simulink model "ZT_VehCtrl_18B_CAN"  (R2018b)
settings: Solver=FixedStepAuto  StartTime=0.0  StopTime=inf  FixedStep=0.005  RelTol=1e-3
InitFcn:
  | mbd_mpc_consistency_checks(bdroot(gcs));
values from neighbouring files (symbols this model uses):
  BatoverTempTh = single(80)    [VCU_INIT.m]
  BRS_PwrValid = single(5)    [VCU_INIT.m]
  BRSEnSpdTh1 = single(10)    [VCU_INIT.m]
  BRSEnSpdTh2 = single(20)    [VCU_INIT.m]
  MCUTempAlarmTh = single (60)    [VCU_INIT.m]
  mps2kmh = single(3.6)    [VCU_INIT.m]
  MtrPwrFac = single(1/9550)    [VCU_INIT.m]
  MtrTempAlarmTh = single (50)    [VCU_INIT.m]
  Padle1Signal1_Th = [PadleSignal1_min,PadleSignal1_max]    [VCU_INIT.m]
  Padle1Signal2_Th = [PadleSignal2_min,PadleSignal2_max]    [VCU_INIT.m]
  PadleSignal1_max = 3.84    [VCU_INIT.m]
  PadleSignal1_min = 0.75    [VCU_INIT.m]
  PadleSignal2_max = 1.92    [VCU_INIT.m]
  PadleSignal2_min = 0.375    [VCU_INIT.m]
  PadleValid = 0.05    [VCU_INIT.m]
  PwrLimFactor = single(0.5)    [VCU_INIT.m]
  Ratio = single(1)    [VCU_INIT.m]
  rpm2mps = single(2*pi/60 * WhlRadius/Ratio)    [VCU_INIT.m]
  SOCLowTh = single(20)    [VCU_INIT.m]
  VehPwrBackwardMax = VehPwrMax * single(0.3)    [VCU_INIT.m]
  VehPwrMax = single(MtrPwrMax * 4)    [VCU_INIT.m]
  VehTrqBackwardMax = VehTrqMax * single(0.3)    [VCU_INIT.m]
  VehTrqMax = single(MtrTrqMax * Ratio *4)    [VCU_INIT.m]
  WhlRadius = single(1)    [VCU_INIT.m]
undefined symbols (not defined in the file or in its folder): Delay_Charge, Delay_Discharge, fifo_0_vect, fifo_1_vect, LQFP, pts1_fifo_0_vect, pts1_fifo_1_vect, pts2_fifo_0_vect, pts2_fifo_1_vect, pts3_fifo_0_vect, pts3_fifo_1_vect, pts4_fifo_0_vect, pts4_fifo_1_vect
libraries: mbd_mpc574x_ec_toolbox x157, canmsglib x74, simulink x38
(part 5 of 12)

== system ZT_VehCtrl_18B_CAN/VehCtrl/EnergyManage ==
  BMS : Inport
  OBC : Inport  Port=2
  HVC : Inport  Port=3
  PDU : Inport  Port=4
  DCDC : Inport  Port=5
  BRS : Inport  Port=6
  DAQ : Inport  Port=7
  Fault : Inport  Port=8
  DrvMtrPwrFb : Inport  Port=9
  VehSpdFb : Inport  Port=10
  Bus Creator : BusCreator  Inputs=2
  Bus Creator1 : BusCreator  Inputs=2
  Bus Creator{4..5,7..10} (6 alike) : BusCreator  Inputs=1
  Bus Creator2 : BusCreator  Inputs=3
  Bus Creator3 : BusCreator  Inputs=3
  Bus Creator6 : BusCreator  Inputs=2
  Bus Selector1 : BusSelector  OutputSignals=BMS_Information2.BMS_ReadySt,BMS_Information2.BMS_PrechargeStatus,BMS Power Infor.BMS_BatteryPower
  Bus Selector2 : BusSelector  OutputSignals=OBC_Charger Status.OBC_StartSt
  Bus Selector4 : BusSelector  OutputSignals=ShutDown,NonBRS,NonOBC
  Bus Selector5 : BusSelector  OutputSignals=ChargeEnSw,AccPadle
  Chart : Stateflow chart  TreatAsAtomicUnit=on
  Data Store Write : DataStoreWrite  DataStoreName=EnergyFlag
  "BMS_OUT " : Outport
  "DCDC_OUT " : Outport  Port=2
  BRS_OUT : Outport  Port=3
  HVC_OUT : Outport  Port=4
  MCU1_OUT : Outport  Port=5
  MCU2_OUT : Outport  Port=6
  ACU_OUT : Outport  Port=7
  PDU_OUT : Outport  Port=8
  TM_OUT : Outport  Port=9
  ISG_OUT : Outport  Port=10
  Ready : Outport  Port=11
  wires:
  BMS/1 -> Bus Selector1/1
  Bus Selector1/1 -> Chart/1(BMS_ReadySt)  "<BMS_ReadySt>"
  OBC/1 -> Bus Selector2/1
  Bus Selector2/1 -> Chart/4(OBC_Start)  "<OBC_StartSt>"
  Bus Selector1/2 -> Chart/2(BMS_PrechargeStatus)  "<BMS_PrechargeStatus>"
  Bus Creator/1 -> "BMS_OUT "/1
  Bus Selector1/3 -> Chart/3(BMS_BatteryPower)  "<BMS_BatteryPower>"
  Chart/1(VCU_PowerOnReq) -> Bus Creator/1  "VCU_PowerOnReq"
  Chart/2(VCU_UrgencyCutOffPowerReq) -> Bus Creator/2  "VCU_UrgencyCutOffPowerReq"
  Chart/11(DcdcCmd) -> Bus Creator1/1  "DcdcCmd"
  Chart/12(DcacEpsCmd) -> Bus Creator1/2  "DcacEpsCmd"
  Bus Creator1/1 -> ACU_OUT/1
  Chart/4(MaxChargePowerLimit) -> Bus Creator2/1  "MaxChargePowerLimit"
  Chart/5(BRS_PowerReq) -> Bus Creator2/2  "BRS_PowerReq"
  Chart/6(OnOffCmd) -> Bus Creator2/3  "OnOffCmd"
  Bus Creator2/1 -> BRS_OUT/1
  Chart/15(VCU_DCCpstRlyCtl) -> Bus Creator3/3  "VCU_DCCpstRlyCtl"
  Chart/14(VCU_HghVtgCtl) -> Bus Creator3/2  "VCU_HghVtgCtl"
  Chart/13(VCU_ShrRlyCtl) -> Bus Creator3/1  "VCU_ShrRlyCtl"
  Chart/9(VCU2OilMotor_ActiveDisCharge) -> Bus Creator5/1  "VCU2OilMotor_ActiveDisCharge"
  Chart/10(VCU2DrvMotor_ActiveDisCharge) -> Bus Creator10/1  "VCU2DrvMotor_ActiveDisCharge"
  Chart/18(TM_Discharge) -> Bus Creator8/1  "TM_Discharge"
  Chart/19(ISG_Discharge) -> Bus Creator9/1  "ISG_Discharge"
  Bus Creator3/1 -> PDU_OUT/1
  Bus Creator6/1 -> HVC_OUT/1
  Chart/7(EDrv1_PowOnCmd) -> Bus Creator6/1  "EDrv1_PowOnCmd"
  Chart/8(EDrv2_PowOnCmd) -> Bus Creator6/2  "EDrv2_PowOnCmd"
  Fault/1 -> Bus Selector4/1
  Bus Selector4/1 -> Chart/8(ShutDown)  "<ShutDown>"
  Bus Selector4/2 -> Chart/9(NonBRS)  "<NonBRS>"
  Bus Selector4/3 -> Chart/10(NonOBC)  "<NonOBC>"
  Chart/16(Ready) -> Bus Creator7/1  "Ready"
  Chart/17(Flag) -> Data Store Write/1  "Flag"
  DAQ/1 -> Bus Selector5/1
  Bus Selector5/1 -> Chart/11(ChargeSig)  "<ChargeEnSw>"
  DrvMtrPwrFb/1 -> Chart/6(PwrCupReq)
  Bus Selector5/2 -> Chart/12(AccPadle)  "<AccPadle>"
  VehSpdFb/1 -> Chart/13(VehSpdFb)
  Chart/3(VCU_DCDC1_En) -> Bus Creator4/1  "VCU_DCDC1_En"
  Bus Creator4/1 -> "DCDC_OUT "/1
  Bus Creator5/1 -> MCU1_OUT/1
  Bus Creator7/1 -> Ready/1
  Bus Creator8/1 -> TM_OUT/1
  Bus Creator9/1 -> ISG_OUT/1
  Bus Creator10/1 -> MCU2_OUT/1

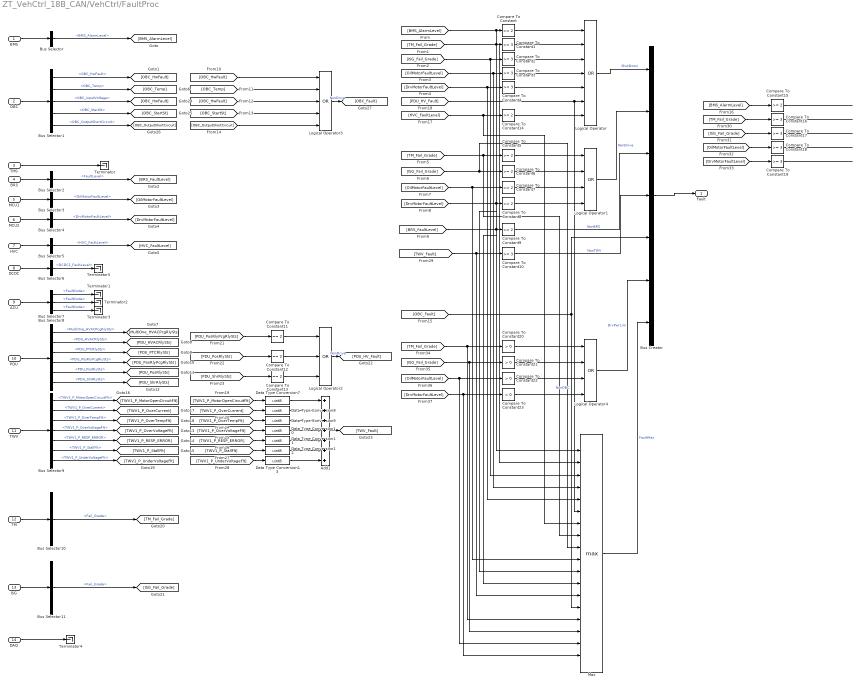
== system ZT_VehCtrl_18B_CAN/VehCtrl/FaultProc ==
  "BMS " : Inport
  "OBC " : Inport  Port=2
  "TMS " : Inport  Port=3
  "BRS " : Inport  Port=4
  "MCU1 " : Inport  Port=5
  MCU2 : Inport  Port=6
  HVC : Inport  Port=7
  DCDC : Inport  Port=8
  ACU : Inport  Port=9
  PDU : Inport  Port=10
  TWV : Inport  Port=11
  TM : Inport  Port=12
  ISG : Inport  Port=13
  DAQ : Inport  Port=14
  Add1 : Sum  Inputs=+++++++
  Bus Creator : BusCreator  Inputs=7
  Bus Selector : BusSelector  OutputSignals=BMS_Information2.BMS_AlarmLevel
  Bus Selector1 : BusSelector  OutputSignals=OBC_Charger Status.OBC_HwFault,OBC_Charger Status.OBC_Temp,OBC_Charger Status.OBC_InputVoltage,OBC_Charger Status.OBC_StartSt,OBC_Charger Status.OBC_OutputShortCircuit
  Bus Selector10 : BusSelector  OutputSignals=TM_MCU_STATUS_2.Fail_Grade
  Bus Selector11 : BusSelector  OutputSignals=ISG_MCU_STATUS_2.Fail_Grade
  Bus Selector2 : BusSelector  OutputSignals=BRS2VCU1.FaultLevel
  Bus Selector3 : BusSelector  OutputSignals=MCU1Msg2.OilMotorFaultLevel
  Bus Selector4 : BusSelector  OutputSignals=MCU2Msg2.DrvMotorFaultLevel
  Bus Selector5 : BusSelector  OutputSignals=HVC4_RlySt.HVC_FaultLevel
  Bus Selector6 : BusSelector  OutputSignals=DCDC1_2.DCDC1_FaultLevel
  Bus Selector7 : BusSelector  OutputSignals=ACU1.FaultCode,ACU2.FaultCode,ACU3.FaultCode
  Bus Selector8 : BusSelector  OutputSignals=PDU_RelaySts.MultiOne_HVACPcgRlySts,PDU_RelaySts.PDU_HVACRlySts,PDU_RelaySts.PDU_PTCRlySts,PDU_RelaySts.PDU_PosRlyPcgRlySts,PDU_RelaySts.PDU_PosRlySts,PDU_RelaySts.PDU_ShrRlySts
  Bus Selector9 : BusSelector  OutputSignals=TWV.TWV1_P_MotorOpenCircuitFlt,TWV.TWV1_P_OverCurrent,TWV.TWV1_P_OverTempFlt,TWV.TWV1_P_OverVoltageFlt,TWV.TWV1_P_RESP_ERROR,TWV.TWV1_P_StallFlt,TWV.TWV1_P_UnderVoltageFlt
  Compare To Constant{,5..9,14..15} (8 alike) : simulink/Logic and Bit Operations/Compare To Constant  relop=>=  const=2  OutDataTypeStr=boolean
  Compare To Constant{1..4,10,16..19} (9 alike) : simulink/Logic and Bit Operations/Compare To Constant  relop=>=  const=3  OutDataTypeStr=boolean
  Compare To Constant11 : simulink/Logic and Bit Operations/Compare To Constant  relop===  const=2  OutDataTypeStr=boolean
  Compare To Constant12 : simulink/Logic and Bit Operations/Compare To Constant  relop===  const=2  OutDataTypeStr=boolean
  Compare To Constant13 : simulink/Logic and Bit Operations/Compare To Constant  relop===  const=2  OutDataTypeStr=boolean
  Compare To Constant{20..23} (4 alike) : simulink/Logic and Bit Operations/Compare To Constant  relop=>  const=0  OutDataTypeStr=boolean
  Data Type Conversion{7..13} (7 alike) : DataTypeConversion  OutDataTypeStr=uint8
  Logical Operator : Logic  Operator=OR  Inputs=7  AllPortsSameDT=off  OutDataTypeStr=boolean
  Logical Operator1 : Logic  Operator=OR  Inputs=4  AllPortsSameDT=off  OutDataTypeStr=boolean
  Logical Operator2 : Logic  Operator=OR  Inputs=3  AllPortsSameDT=off  OutDataTypeStr=boolean
  Logical Operator3 : Logic  Operator=OR  Inputs=5  AllPortsSameDT=off  OutDataTypeStr=boolean
  Logical Operator4 : Logic  Operator=OR  Inputs=4  AllPortsSameDT=off  OutDataTypeStr=boolean
  Max : MinMax  Function=max  Inputs=18
  Terminator{,1..5} (6 alike) : Terminator
  "Fault " : Outport
  wires:
  "BMS "/1 -> Bus Selector/1
  Bus Selector/1 -> [BMS_AlarmLevel]  "<BMS_AlarmLevel>"
  "OBC "/1 -> Bus Selector1/1
  Bus Selector1/1 -> [OBC_HwFault]  "<OBC_HwFault>"
  "TMS "/1 -> Terminator/1
  "BRS "/1 -> Bus Selector2/1
  "MCU1 "/1 -> Bus Selector3/1
  Bus Selector3/1 -> [OilMotorFaultLevel]  "<OilMotorFaultLevel>"
  Bus Selector2/1 -> [BRS_FaultLevel]  "<FaultLevel>"
  MCU2/1 -> Bus Selector4/1
  Bus Selector4/1 -> [DrvMotorFaultLevel]  "<DrvMotorFaultLevel>"
  HVC/1 -> Bus Selector5/1
  Bus Selector5/1 -> [HVC_FaultLevel]  "<HVC_FaultLevel>"
  DCDC/1 -> Bus Selector6/1
  Bus Selector6/1 -> Terminator5/1  "<DCDC1_FaultLevel>"
  ACU/1 -> Bus Selector7/1
  Bus Selector7/1 -> Terminator1/1  "<FaultCode>"
  Bus Selector7/2 -> Terminator2/1  "<FaultCode>"
  Bus Selector7/3 -> Terminator3/1  "<FaultCode>"
  PDU/1 -> Bus Selector8/1
  TWV/1 -> Bus Selector9/1
  TM/1 -> Bus Selector10/1
  ISG/1 -> Bus Selector11/1
  DAQ/1 -> Terminator4/1
  Bus Selector8/1 -> [MultiOne_HVACPcgRlySts]  "<MultiOne_HVACPcgRlySts>"
  Bus Selector8/2 -> [PDU_HVACRlySts]  "<PDU_HVACRlySts>"
  Bus Selector8/3 -> [PDU_PTCRlySts]  "<PDU_PTCRlySts>"
  Bus Selector8/4 -> [PDU_PosRlyPcgRlySts]  "<PDU_PosRlyPcgRlySts>"
  Bus Selector8/5 -> [PDU_PosRlySts]  "<PDU_PosRlySts>"
  Bus Selector8/6 -> [PDU_ShrRlySts]  "<PDU_ShrRlySts>"
  Bus Selector9/1 -> [TWV1_P_MotorOpenCircuitFlt]  "<TWV1_P_MotorOpenCircuitFlt>"
  Bus Selector9/2 -> [TWV1_P_OverCurrent]  "<TWV1_P_OverCurrent>"
  Bus Selector9/3 -> [TWV1_P_OverTempFlt]  "<TWV1_P_OverTempFlt>"
  Bus Selector9/4 -> [TWV1_P_OverVoltageFlt]  "<TWV1_P_OverVoltageFlt>"
  Bus Selector9/5 -> [TWV1_P_RESP_ERROR]  "<TWV1_P_RESP_ERROR>"
  Bus Selector9/6 -> [TWV1_P_StallFlt]  "<TWV1_P_StallFlt>"
  Bus Selector9/7 -> [TWV1_P_UnderVoltageFlt]  "<TWV1_P_UnderVoltageFlt>"
  Bus Selector10/1 -> [TM_Fail_Grade]  "<Fail_Grade>"
  Bus Selector11/1 -> [ISG_Fail_Grade]  "<Fail_Grade>"
  [BMS_AlarmLevel] -> Max/1, Compare To Constant/1
  [TM_Fail_Grade] -> Max/2, Compare To Constant1/1
  [ISG_Fail_Grade] -> Compare To Constant2/1, Max/3
  [DrvMotorFaultLevel] -> Compare To Constant4/1, Max/5
  [OilMotorFaultLevel] -> Compare To Constant3/1, Max/4
  Compare To Constant/1 -> Logical Operator/1
  Compare To Constant1/1 -> Logical Operator/2
  Compare To Constant2/1 -> Logical Operator/3
  Compare To Constant3/1 -> Logical Operator/4
  Compare To Constant4/1 -> Logical Operator/5
  Logical Operator/1 -> Bus Creator/1  "ShutDown"
  Bus Creator/1 -> "Fault "/1
  Compare To Constant8/1 -> Logical Operator1/4
  Compare To Constant7/1 -> Logical Operator1/3
  Compare To Constant6/1 -> Logical Operator1/2
  [OilMotorFaultLevel] -> Max/10, Compare To Constant7/1
  [DrvMotorFaultLevel] -> Max/11, Compare To Constant8/1
  [ISG_Fail_Grade] -> Max/9, Compare To Constant6/1
  [TM_Fail_Grade] -> Compare To Constant5/1, Max/8
  Compare To Constant5/1 -> Logical Operator1/1
  Logical Operator1/1 -> Bus Creator/2  "NonDrive"
  [BRS_FaultLevel] -> Max/12, Compare To Constant9/1
  Compare To Constant9/1 -> Bus Creator/3  "NonBRS"
  Compare To Constant10/1 -> Bus Creator/4  "NonTWV"
  [PDU_PosRlyPcgRlySts] -> Compare To Constant11/1
  [PDU_PosRlySts] -> Compare To Constant12/1
  [PDU_ShrRlySts] -> Compare To Constant13/1
  Compare To Constant11/1 -> Logical Operator2/1
  Compare To Constant12/1 -> Logical Operator2/2
  Compare To Constant13/1 -> Logical Operator2/3
  Logical Operator2/1 -> [PDU_HV_Fault]  "NonDrive"
  [PDU_HV_Fault] -> Max/6, Logical Operator/6
  [HVC_FaultLevel] -> Compare To Constant14/1, Max/7
  Compare To Constant14/1 -> Logical Operator/7
  Data Type Conversion13/1 -> Add1/7
  Data Type Conversion12/1 -> Add1/6
  Data Type Conversion11/1 -> Add1/5
  Data Type Conversion10/1 -> Add1/4
  Data Type Conversion9/1 -> Add1/3
  Data Type Conversion8/1 -> Add1/2
  Data Type Conversion7/1 -> Add1/1
  [TWV1_P_OverCurrent] -> Data Type Conversion8/1
  [TWV1_P_OverTempFlt] -> Data Type Conversion9/1
  [TWV1_P_OverVoltageFlt] -> Data Type Conversion10/1
  [TWV1_P_RESP_ERROR] -> Data Type Conversion11/1
  [TWV1_P_StallFlt] -> Data Type Conversion12/1
  [TWV1_P_UnderVoltageFlt] -> Data Type Conversion13/1
  [TWV1_P_MotorOpenCircuitFlt] -> Data Type Conversion7/1
  Add1/1 -> [TWV_Fault]
  [TWV_Fault] -> Compare To Constant10/1, Max/13
  Bus Selector1/2 -> [OBC_Temp]  "<OBC_Temp>"
  Bus Selector1/3 -> [OBC_HwFault]  "<OBC_InputVoltage>"
  Bus Selector1/4 -> [OBC_StartSt]  "<OBC_StartSt>"
  Bus Selector1/5 -> [OBC_OutputShortCircuit]  "<OBC_OutputShortCircuit>"
  [OBC_HwFault] -> Logical Operator3/1
  [OBC_Temp] -> Logical Operator3/2
  [OBC_HwFault] -> Logical Operator3/3
  [OBC_StartSt] -> Logical Operator3/4
  [OBC_OutputShortCircuit] -> Logical Operator3/5
  Logical Operator3/1 -> [OBC_Fault]  "NonDrive"
  [OBC_Fault] -> Bus Creator/5, Max/14  "NonOBC"
  Compare To Constant19/1 -> ?
  Compare To Constant18/1 -> ?
  Compare To Constant17/1 -> ?
  Compare To Constant16/1 -> ?
  Compare To Constant15/1 -> ?
  [OilMotorFaultLevel] -> Compare To Constant18/1
  [DrvMotorFaultLevel] -> Compare To Constant19/1
  [ISG_Fail_Grade] -> Compare To Constant17/1
  [TM_Fail_Grade] -> Compare To Constant16/1
  [BMS_AlarmLevel] -> Compare To Constant15/1
  Compare To Constant20/1 -> Logical Operator4/1
  [TM_Fail_Grade] -> Compare To Constant20/1, Max/15
  [ISG_Fail_Grade] -> Compare To Constant21/1, Max/16
  [DrvMotorFaultLevel] -> Compare To Constant23/1, Max/18
  [OilMotorFaultLevel] -> Max/17, Compare To Constant22/1
  Compare To Constant21/1 -> Logical Operator4/2
  Compare To Constant22/1 -> Logical Operator4/3
  Compare To Constant23/1 -> Logical Operator4/4
  Logical Operator4/1 -> Bus Creator/6  "DrvPwrLim"
  Max/1 -> Bus Creator/7  "FaultMax"

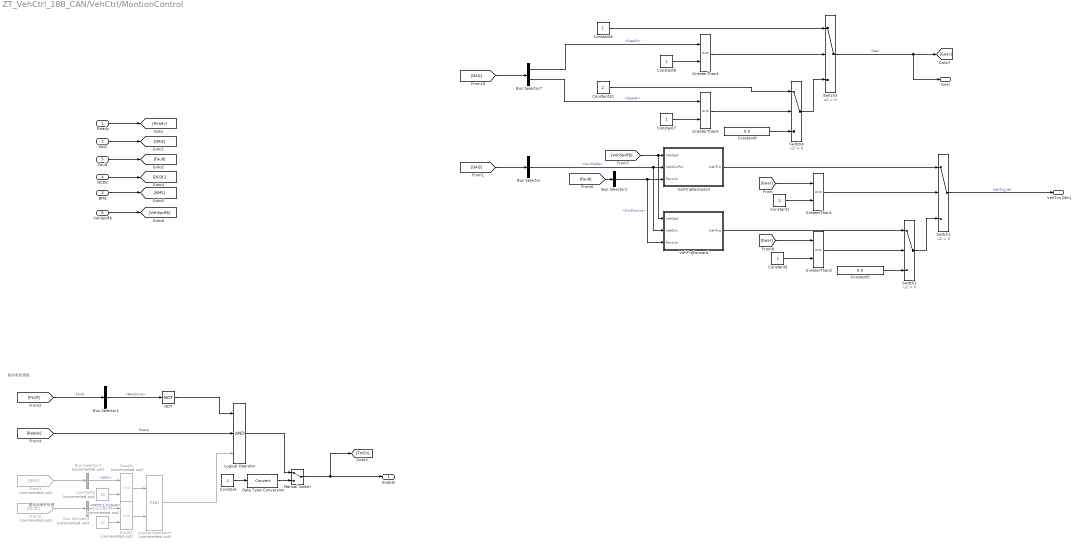
== system ZT_VehCtrl_18B_CAN/VehCtrl/MontionControl ==
  note: 驱动电机使能
  note: 蓄电池保护处理
  Ready : Inport
  DAQ : Inport  Port=2
  BMS : Inport  Port=3
  DCDC : Inport  Port=4
  Fault : Inport  Port=5
  VehSpdFb : Inport  Port=6
  Bus Selector : BusSelector  OutputSignals=AccPadle
  Bus Selector1 : BusSelector  OutputSignals=NonDrive
  Bus Selector2 : BusSelector  OutputSignals=DrvPwrLim
  Bus Selector3 : BusSelector  Commented=on  OutputSignals=BMS_Information1.SOC
  Bus Selector4 : BusSelector  Commented=on  OutputSignals=DCDC1_1.DCDC1_OutVolt
  Bus Selector7 : BusSelector  OutputSignals=GearD,GearR
  Constant : Constant
  Constant1 : Constant  Value=2  OutDataTypeStr=single
  Constant10 : Constant  Value=2  OutDataTypeStr=single
  Constant2 : Constant  Commented=on  Value=30  OutDataTypeStr=boolean
  Constant3 : Constant  OutDataTypeStr=single
  Constant4 : Constant  Commented=on  Value=22  OutDataTypeStr=boolean
  Constant5 : Constant  Value=0.0  OutDataTypeStr=single
  Constant6 : Constant  OutDataTypeStr=boolean
  Constant7 : Constant  OutDataTypeStr=boolean
  Constant8 : Constant  Value=0.0  OutDataTypeStr=single
  Constant9 : Constant  OutDataTypeStr=int8
  Data Type Conversion : DataTypeConversion
  Equal1 : RelationalOperator  Commented=on  OutDataTypeStr=boolean  RndMeth=Simplest
  Equal2 : RelationalOperator  Commented=on  OutDataTypeStr=boolean  RndMeth=Simplest
  From3 : From  Commented=on  GotoTag=BMS
  From5 : From  Commented=on  GotoTag=DCDC
  GreaterThan{1..2,4..5} (4 alike) : RelationalOperator  Operator===  OutDataTypeStr=boolean  RndMeth=Simplest
  Logical Operator : Logic  Inputs=3  AllPortsSameDT=off  OutDataTypeStr=boolean
  Logical Operator1 : Logic  Commented=on  AllPortsSameDT=off  OutDataTypeStr=boolean
  Manual Switch : ManualSwitch
  NOT : Logic  Operator=NOT  IconShape=distinctive  AllPortsSameDT=off  OutDataTypeStr=boolean
  Switch{1..4} (4 alike) : Switch  Criteria=u2 > Threshold
  VehTrqBackward : Subsystem
  VehTrqForward : Subsystem
  Enable : Outport
  VehTrq [Nm] : Outport  Port=2
  Gear : Outport  Port=3
  wires:
  Ready/1 -> [Ready]
  DAQ/1 -> [DAQ]
  [DAQ] -> Bus Selector/1
  Fault/1 -> [Fault]
  Bus Selector/1 -> VehTrqForward/2(VehDrv), VehTrqBackward/2(VehDrvPct)  "<AccPadle>"
  [Fault] -> Bus Selector1/1  "Fault"
  [Ready] -> Logical Operator/2  "Ready"
  Bus Selector4/1 -> Equal2/1  "<DCDC1_OutVolt>"
  Logical Operator/1 -> Manual Switch/1
  Equal2/1 -> Logical Operator1/2
  Data Type Conversion/1 -> Manual Switch/2
  Constant4/1 -> Equal2/2
  From5/1 -> Bus Selector4/1
  From3/1 -> Bus Selector3/1
  Bus Selector3/1 -> Equal1/1  "<SOC>"
  Logical Operator1/1 -> Logical Operator/3
  Manual Switch/1 -> [TmEn], Enable/1
  Equal1/1 -> Logical Operator1/1
  NOT/1 -> Logical Operator/1
  Constant/1 -> Data Type Conversion/1
  Bus Selector1/1 -> NOT/1  "<NonDrive>"
  Constant2/1 -> Equal1/2
  BMS/1 -> [BMS]
  DCDC/1 -> [DCDC]
  VehTrqForward/1(VehTrq) -> Switch2/1
  GreaterThan1/1 -> Switch1/2
  VehTrqBackward/1(VehTrq) -> Switch1/1
  Constant5/1 -> Switch2/3
  GreaterThan2/1 -> Switch2/2
  Constant1/1 -> GreaterThan1/2
  Switch2/1 -> Switch1/3
  Constant3/1 -> GreaterThan2/2
  Switch1/1 -> VehTrq [Nm]/1  "VehTrq_ter"
  [Fault] -> Bus Selector2/1
  Bus Selector2/1 -> VehTrqForward/3(PwrLim), VehTrqBackward/3(PwrLim)  "<DrvPwrLim>"
  VehSpdFb/1 -> [VehSpdFb]
  [VehSpdFb] -> VehTrqForward/1(VehSpd), VehTrqBackward/1(VehSpd)
  [DAQ] -> Bus Selector7/1
  Switch3/1 -> Gear/1, [Gear]  "Gear"
  Constant7/1 -> GreaterThan5/2
  Switch4/1 -> Switch3/3
  Constant6/1 -> GreaterThan4/2
  GreaterThan5/1 -> Switch4/2
  Constant8/1 -> Switch4/3
  Constant9/1 -> Switch3/1
  GreaterThan4/1 -> Switch3/2
  Constant10/1 -> Switch4/1
  Bus Selector7/1 -> GreaterThan4/1  "<GearD>"
  Bus Selector7/2 -> GreaterThan5/1  "<GearR>"
  [Gear] -> GreaterThan1/1
  [Gear] -> GreaterThan2/1

== system ZT_VehCtrl_18B_CAN/VehCtrl/SpdCalc ==
  MCU2 : Inport
  TM : Inport  Port=2
  MCU1 : Inport  Port=3
  ISG : Inport  Port=4
  Abs{1..4} (4 alike) : Abs
  Add{,1..3} (4 alike) : Sum
  Bus Selector : BusSelector  OutputSignals=MCU2Msg1.DrvMotorSpd,MCU2Msg1.DrvMotorTrq
  Bus Selector1 : BusSelector  OutputSignals=TM_MCU_STATUS_1.Motor_Speed,TM_MCU_STATUS_1.Motor_Torque
  Bus Selector2 : BusSelector  OutputSignals=MCU1Msg1.OilMotorSpd,MCU1Msg1.OilMotorTrq
  Bus Selector3 : BusSelector  OutputSignals=ISG_MCU_STATUS_1.Motor_Speed,ISG_MCU_STATUS_1.Motor_Torque
  Constant : Constant  Value=rpm2mps
  Gain : Gain  Gain=0.5
  Gain1 : Gain  Gain=MtrPwrFac
  Gain2 : Gain  Gain=MtrPwrFac
  Gain3 : Gain  Gain=Ratio
  Product{,1..4} (5 alike) : Product
  VehSpdFb : Outport
  "VehTrqFb " : Outport  Port=2
  "DrvMtrPwrFb " : Outport  Port=3
  "OilMtrPwrFb " : Outport  Port=4
  wires:
  MCU2/1 -> Bus Selector/1
  TM/1 -> Bus Selector1/1
  MCU1/1 -> Bus Selector2/1
  ISG/1 -> Bus Selector3/1
  Bus Selector1/1 -> Abs1/1  "<Motor_Speed>"
  Bus Selector3/1 -> Abs3/1  "<Motor_Speed>"
  Bus Selector/2 -> Add2/1, Product1/2  "<DrvMotorTrq>"
  Abs1/1 -> Product2/2, Add/2
  Add/1 -> Gain/1
  Product/1 -> VehSpdFb/1
  Gain/1 -> Product/1
  Constant/1 -> Product/2
  Abs2/1 -> Product1/1, Add/1
  Product1/1 -> Add1/1
  Product2/1 -> Add1/2
  Bus Selector1/2 -> Add2/2, Product2/1  "<Motor_Torque>"
  Add1/1 -> Gain1/1
  Gain1/1 -> "DrvMtrPwrFb "/1
  Add2/1 -> Gain3/1
  Bus Selector/1 -> Abs2/1  "<DrvMotorSpd>"
  Bus Selector2/1 -> Abs4/1  "<OilMotorSpd>"
  Bus Selector2/2 -> Product3/2  "<OilMotorTrq>"
  Bus Selector3/2 -> Product4/2  "<Motor_Torque>"
  Add3/1 -> Gain2/1
  Abs3/1 -> Product4/1
  Product3/1 -> Add3/1
  Gain2/1 -> "OilMtrPwrFb "/1
  Product4/1 -> Add3/2
  Abs4/1 -> Product3/1
  Gain3/1 -> "VehTrqFb "/1

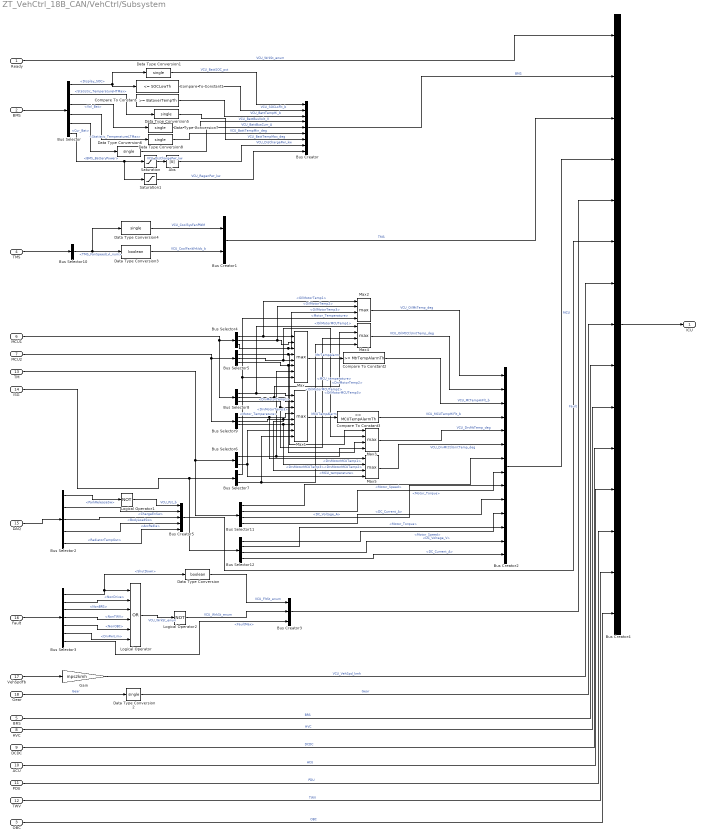
== system ZT_VehCtrl_18B_CAN/VehCtrl/Subsystem ==
  Ready : Inport
  BMS : Inport  Port=2
  OBC : Inport  Port=3
  TMS : Inport  Port=4
  BRS : Inport  Port=5
  MCU1 : Inport  Port=6
  MCU2 : Inport  Port=7
  HVC : Inport  Port=8
  DCDC : Inport  Port=9
  ACU : Inport  Port=10
  PDU : Inport  Port=11
  TWV : Inport  Port=12
  TM : Inport  Port=13
  ISG : Inport  Port=14
  DAQ : Inport  Port=15
  Fault : Inport  Port=16
  VehSpdFb : Inport  Port=17
  Gear : Inport  Port=18
  Abs : Abs
  Bus Creator : BusCreator  Inputs=9
  Bus Creator1 : BusCreator  Inputs=2
  Bus Creator2 : BusCreator  Inputs=14
  Bus Creator3 : BusCreator  Inputs=3
  Bus Creator4 : BusCreator  Inputs=15
  Bus Creator5 : BusCreator  Inputs=5
  Bus Selector : BusSelector  OutputSignals=BMS_Information1.Display_SOC,BMS Statistic_Temperature of Battery.Statistic_TemperatureHTMax,BMS_Information1.Vol_Bat,BMS Statistic_Temperature of Battery.Statistic_TemperatureLTMax,BMS_Information1.Cur_Bat,BMS Power Infor.BMS_BatteryPower
  Bus Selector10 : BusSelector  OutputSignals=TMS2VCU.TMS_FanSpeedLvl_num
  Bus Selector11 : BusSelector  OutputSignals=TM_MCU_STATUS_1.Motor_Speed,TM_MCU_STATUS_1.Motor_Torque,TM_MCU_STATUS_3.DC_Voltage_A,TM_MCU_STATUS_3.DC_Current_A
  Bus Selector12 : BusSelector  OutputSignals=ISG_MCU_STATUS_1.Motor_Speed,ISG_MCU_STATUS_1.Motor_Torque,ISG_MCU_STATUS_3.DC_Voltage_V,ISG_MCU_STATUS_3.DC_Current_A
  Bus Selector2 : BusSelector  OutputSignals=ParkReleaseSw,ChargeEnSw,BodyLoadSw,AccPadle,RadiatorTempOut
  Bus Selector3 : BusSelector  OutputSignals=ShutDown,NonDrive,NonBRS,NonTWV,NonOBC,DrvPwrLim,FaultMax
  Bus Selector4 : BusSelector  OutputSignals=MCU1Msg3.OilMotorTemp1,MCU1Msg3.OilMotorTemp2,MCU1Msg3.OilMotorTemp3
  Bus Selector5 : BusSelector  OutputSignals=MCU2Msg3.DrvMotorTemp1,MCU2Msg3.DrvMotorTemp2,MCU2Msg3.DrvMotorTemp3
  Bus Selector6 : BusSelector  OutputSignals=TM_MCU_STATUS_2.Motor_Temperature,TM_MCU_STATUS_2.MCU_temperature
  Bus Selector7 : BusSelector  OutputSignals=ISG_MCU_STATUS_2.Motor_Temperature,ISG_MCU_STATUS_2.MCU_temperature
  Bus Selector8 : BusSelector  OutputSignals=MCU1Msg3.OilMotorMCUTemp1,MCU1Msg3.OilMotorMCUTemp2,MCU1Msg3.OilMotorMCUTemp3
  Bus Selector9 : BusSelector  OutputSignals=MCU2Msg3.DrvMotorMCUTemp1,MCU2Msg3.DrvMotorMCUTemp2,MCU2Msg3.DrvMotorMCUTemp3
  Compare To Constant : simulink/Logic and Bit Operations/Compare To Constant  relop=>=  const=BatoverTempTh  OutDataTypeStr=boolean
  Compare To Constant1 : simulink/Logic and Bit Operations/Compare To Constant  relop=<=  const=SOCLowTh  OutDataTypeStr=boolean
  Compare To Constant2 : simulink/Logic and Bit Operations/Compare To Constant  relop=>=  const=MtrTempAlarmTh  OutDataTypeStr=boolean
  Compare To Constant3 : simulink/Logic and Bit Operations/Compare To Constant  relop=>=  const=MCUTempAlarmTh  OutDataTypeStr=boolean
  Data Type Conversion : DataTypeConversion  OutDataTypeStr=boolean
  Data Type Conversion{1..2,4..8} (7 alike) : DataTypeConversion  OutDataTypeStr=single
  Data Type Conversion3 : DataTypeConversion  OutDataTypeStr=boolean
  Gain : Gain  Gain=mps2kmh
  Logical Operator : Logic  Operator=OR  Inputs=6  AllPortsSameDT=off  OutDataTypeStr=boolean
  Logical Operator1 : Logic  Operator=NOT  AllPortsSameDT=off  OutDataTypeStr=boolean
  Logical Operator2 : Logic  Operator=NOT  AllPortsSameDT=off  OutDataTypeStr=boolean
  Max : MinMax  Function=max  Inputs=8
  Max1 : MinMax  Function=max  Inputs=8
  Max{2..5} (4 alike) : MinMax  Function=max  Inputs=4
  Saturation : Saturate  UpperLimit=0  LowerLimit=-1000
  Saturation1 : Saturate  UpperLimit=+1000  LowerLimit=0
  ICU : Outport
  wires:
  BMS/1 -> Bus Selector/1
  Bus Selector/1 -> Compare To Constant1/1, Data Type Conversion1/1  "<Display_SOC>"
  Bus Selector/2 -> Data Type Conversion5/1, Compare To Constant/1  "<Statistic_TemperatureHTMax>"
  Bus Selector/3 -> Data Type Conversion7/1  "<Vol_Bat>"
  Bus Selector/4 -> Data Type Conversion8/1  "<Statistic_TemperatureLTMax>"
  OBC/1 -> Bus Creator4/15  "OBC"
  DAQ/1 -> Bus Selector2/1
  Fault/1 -> Bus Selector3/1
  Bus Selector3/1 -> Data Type Conversion/1, Logical Operator/1  "<ShutDown>"
  Bus Selector3/2 -> Logical Operator/2  "<NonDrive>"
  Bus Selector3/3 -> Logical Operator/3  "<NonBRS>"
  Bus Selector3/4 -> Logical Operator/4  "<NonTWV>"
  Bus Selector3/5 -> Logical Operator/5  "<NonOBC>"
  Bus Selector3/6 -> Logical Operator/6  "<DrvPwrLim>"
  Logical Operator/1 -> Logical Operator2/1  "VCU_WrkSt_enum"
  Bus Selector2/1 -> Logical Operator1/1  "<ParkReleaseSw>"
  Logical Operator1/1 -> Bus Creator5/1  "VCU_Pst_b"
  Compare To Constant1/1 -> Bus Creator/2  "VCU_SOCLoFlt_b"
  Data Type Conversion/1 -> Bus Creator3/1  "VCU_FltSt_enum"
  Logical Operator2/1 -> Bus Creator3/2  "VCU_WrkSt_enum"
  Ready/1 -> Bus Creator4/1  "VCU_WrkSt_enum"
  VehSpdFb/1 -> Gain/1
  Gain/1 -> Bus Creator4/7  "VCU_VehSpd_kmh"
  Data Type Conversion1/1 -> Bus Creator/1  "VCU_BattSOC_pct"
  Gear/1 -> Data Type Conversion2/1  "Gear"
  Data Type Conversion2/1 -> Bus Creator4/8  "Gear"
  Bus Selector2/2 -> Bus Creator5/2  "<ChargeEnSw>"
  MCU1/1 -> Bus Selector8/1, Bus Selector4/1
  MCU2/1 -> Bus Selector9/1, Bus Selector5/1
  ISG/1 -> Bus Selector12/1, Bus Selector7/1
  Bus Selector4/1 -> Max2/1, Max/1  "<OilMotorTemp1>"
  Bus Selector4/2 -> Max2/2, Max/2  "<OilMotorTemp2>"
  Bus Selector4/3 -> Max2/3, Max/3  "<OilMotorTemp3>"
  Bus Selector5/1 -> Max3/1, Max/4  "<DrvMotorTemp1>"
  Bus Selector5/2 -> Max3/2, Max/5  "<DrvMotorTemp2>"
  Bus Selector5/3 -> Max3/3, Max/6  "<DrvMotorTemp3>"
  TM/1 -> Bus Selector11/1, Bus Selector6/1
  Bus Selector6/1 -> Max3/4, Max/7  "<Motor_Temperature>"
  Bus Selector7/1 -> Max2/4, Max/8  "<Motor_Temperature>"
  Max/1 -> Compare To Constant2/1  "MtrTempAlarm"
  Bus Selector8/1 -> Max4/1, Max1/1  "<OilMotorMCUTemp1>"
  Bus Selector8/2 -> Max4/2, Max1/2  "<OilMotorMCUTemp2>"
  Bus Selector8/3 -> Max4/3, Max1/3  "<OilMotorMCUTemp3>"
  Bus Selector9/1 -> Max5/1, Max1/4  "<DrvMotorMCUTemp1>"
  Bus Selector9/2 -> Max5/3, Max1/5  "<DrvMotorMCUTemp2>"
  Bus Selector9/3 -> Max5/2, Max1/6  "<DrvMotorMCUTemp3>"
  Bus Selector6/2 -> Max5/4, Max1/7  "<MCU_temperature>"
  Bus Selector7/2 -> Max4/4, Max1/8  "<MCU_temperature>"
  Max1/1 -> Compare To Constant3/1  "MCUTempAlarm"
  Compare To Constant2/1 -> Bus Creator2/3  "VCU_MtTempHiFlt_b"
  Compare To Constant3/1 -> Bus Creator2/4  "VCU_MCUTempHiFlt_b"
  Bus Selector2/3 -> Bus Creator5/3  "<BodyLoadSw>"
  TMS/1 -> Bus Selector10/1
  Bus Selector10/1 -> Data Type Conversion4/1, Data Type Conversion3/1  "<TMS_FanSpeedLvl_num>"
  Data Type Conversion3/1 -> Bus Creator1/2  "VCU_CoolFanWrkIdc_b"
  Data Type Conversion4/1 -> Bus Creator1/1  "VCU_CoolSysFanPWM"
  Bus Selector/5 -> Data Type Conversion6/1  "<Cur_Bat>"
  Max2/1 -> Bus Creator2/1  "VCU_OilMtTemp_deg"
  Max4/1 -> Bus Creator2/2  "VCU_OilMtCtlUnitTemp_deg"
  Bus Selector2/4 -> Bus Creator5/4  "<AccPadle>"
  Bus Selector2/5 -> Bus Creator5/5  "<RadiatorTempOut>"
  Max3/1 -> Bus Creator2/5  "VCU_DrvMtTemp_deg"
  Max5/1 -> Bus Creator2/6  "VCU_DrvMtCtlUnitTemp_deg"
  Data Type Conversion5/1 -> Bus Creator/7  "VCU_BattTempMax_deg"
  Bus Selector11/1 -> Bus Creator2/7  "<Motor_Speed>"
  Bus Selector11/2 -> Bus Creator2/8  "<Motor_Torque>"
  Bus Selector11/3 -> Bus Creator2/9  "<DC_Voltage_A>"
  Bus Selector11/4 -> Bus Creator2/10  "<DC_Current_A>"
  Bus Selector/6 -> Saturation1/1, Saturation/1  "<BMS_BatteryPower>"
  Saturation/1 -> Abs/1  "VCU_DisChargePwr_kw"
  Saturation1/1 -> Bus Creator/9  "VCU_RegenPwr_kw"
  Abs/1 -> Bus Creator/8  "VCU_DisChargePwr_kw"
  Bus Creator/1 -> Bus Creator4/2  "BMS"
  Bus Creator1/1 -> Bus Creator4/3  "TMS"
  Bus Selector12/1 -> Bus Creator2/11  "<Motor_Speed>"
  Bus Selector12/2 -> Bus Creator2/12  "<Motor_Torque>"
  Bus Selector12/3 -> Bus Creator2/13  "<DC_Voltage_V>"
  Bus Selector12/4 -> Bus Creator2/14  "<DC_Current_A>"
  Bus Creator2/1 -> Bus Creator4/4  "MCU"
  Bus Creator3/1 -> Bus Creator4/5  "Fault"
  BRS/1 -> Bus Creator4/9  "BRS"
  HVC/1 -> Bus Creator4/10  "HVC"
  DCDC/1 -> Bus Creator4/11  "DCDC"
  ACU/1 -> Bus Creator4/12  "ACU"
  PDU/1 -> Bus Creator4/13  "PDU"
  TWV/1 -> Bus Creator4/14  "TWV"
  Bus Creator4/1 -> ICU/1
  Bus Creator5/1 -> Bus Creator4/6
  Compare To Constant/1 -> Bus Creator/3  "VCU_BattTempHi_b"
  Bus Selector3/7 -> Bus Creator3/3  "<FaultMax>"
  Data Type Conversion6/1 -> Bus Creator/5  "VCU_BattBusCurr_A"
  Data Type Conversion7/1 -> Bus Creator/4  "VCU_BattBusVolt_V"
  Data Type Conversion8/1 -> Bus Creator/6  "VCU_BattTempMin_deg"

== system ZT_VehCtrl_18B_CAN/VehCtrl/TempertureControl ==
  BMS : Inport
  OBC : Inport  Port=2
  MCU1 : Inport  Port=3
  MCU2 : Inport  Port=4
  TM : Inport  Port=5
  ISG : Inport  Port=6
  Bus Selector : BusSelector  OutputSignals=BMS Statistic_Temperature of Battery.Statistic_TemperatureHTMax
  Bus Selector1 : BusSelector  OutputSignals=OBC_Charger Status.OBC_Temp
  VCU_FanSpeedLvl_num : Outport
  VCU_TWV1_P_PosSet : Outport  Port=2
  wires:
  BMS/1 -> [BMS]
  OBC/1 -> [OBC]
  MCU1/1 -> [MCU1]
  MCU2/1 -> [MCU2]
  ISG/1 -> [ISG]
  TM/1 -> [TM]
  [BMS] -> Bus Selector/1
  [OBC] -> Bus Selector1/1
  Bus Selector/1 -> ?  "<Statistic_TemperatureHTMax>"
  Bus Selector1/1 -> ?  "<OBC_Temp>"

== system ZT_VehCtrl_18B_CAN/Initialization & SPI timer1/CS1 LS/Subsystem ==
  Data Store Read : DataStoreRead  DataStoreName=SPIO_CS1_InitFlg
  Merge : Merge  Inputs=3
  Merge1 : Merge  Inputs=3
  SPI_en : Subsystem  TreatAsAtomicUnit=on
  Switch Case : SwitchCase  CaseConditions={1,2,3}  ShowDefaultCase=off
  "clear " : Subsystem  TreatAsAtomicUnit=on
  confi_enbit : Subsystem  TreatAsAtomicUnit=on
  Out1 : Outport
  Out2 : Outport  Port=2
  wires:
  confi_enbit/1(Out1) -> Merge/3
  SPI_en/1(Out1) -> Merge/2
  "clear "/2(Out2) -> Merge1/1
  confi_enbit/2(Out2) -> Merge1/3
  "clear "/1(Out1) -> Merge/1
  Switch Case/1 -> "clear "/Action
  Switch Case/3 -> confi_enbit/Action
  Merge1/1 -> Out2/1
  Switch Case/2 -> SPI_en/Action
  SPI_en/2(Out2) -> Merge1/2
  Data Store Read/1 -> Switch Case/1
  Merge/1 -> Out1/1

== system ZT_VehCtrl_18B_CAN/Initialization & SPI timer1/CS3 LS/Subsystem ==
  In1 : Inport
  In2 : Inport  Port=2
  A组配置 : Subsystem  TreatAsAtomicUnit=on
  B组配置 : Subsystem  TreatAsAtomicUnit=on
  Data Store Read : DataStoreRead  DataStoreName=SPI3_CTRL1
  Merge : Merge  Inputs=3
  Merge1 : Merge  Inputs=3
  Switch Case : SwitchCase  CaseConditions={1,2,3}  ShowDefaultCase=off
  Out1 : Outport
  Out2 : Outport  Port=2
  Out3 : Outport  Port=3
  wires:
  Switch Case/2 -> B组配置/Action
  Merge1/1 -> Out3/1
  A组配置/2(Out2) -> Merge1/1
  In2/1 -> Merge1/3
  Data Store Read/1 -> Switch Case/1
  B组配置/1(Out1) -> Merge/2
  Merge/1 -> Out2/1
  Switch Case/3 -> Out1/1
  A组配置/1(Out1) -> Merge/1
  B组配置/2(Out2) -> Merge1/2
  Switch Case/1 -> A组配置/Action
  In1/1 -> Merge/3

== system ZT_VehCtrl_18B_CAN/Initialization & SPI timer1/CS5 LS/Subsystem ==
  Data Store Read : DataStoreRead  DataStoreName=SPIO_CS1_InitFlg
  Merge : Merge  Inputs=3
  Merge1 : Merge  Inputs=3
  SPI_en : Subsystem  TreatAsAtomicUnit=on
  Switch Case : SwitchCase  CaseConditions={1,2,3}  ShowDefaultCase=off
  "clear " : Subsystem  TreatAsAtomicUnit=on
  confi_enbit : Subsystem  TreatAsAtomicUnit=on
  Out1 : Outport
  Out2 : Outport  Port=2
  wires:
  confi_enbit/1(Out1) -> Merge/3
  SPI_en/1(Out1) -> Merge/2
  "clear "/2(Out2) -> Merge1/1
  confi_enbit/2(Out2) -> Merge1/3
  "clear "/1(Out1) -> Merge/1
  Switch Case/1 -> "clear "/Action
  Switch Case/3 -> confi_enbit/Action
  Merge1/1 -> Out2/1
  Switch Case/2 -> SPI_en/Action
  SPI_en/2(Out2) -> Merge1/2
  Data Store Read/1 -> Switch Case/1
  Merge/1 -> Out1/1

== system ZT_VehCtrl_18B_CAN/SPI_EEPROM/SPI_write/SPI_enable ==
  Action Port : ActionPort
  Constant1 : Constant  Value=2
  Data Store Write : DataStoreWrite  DataStoreName=Write_Ctrl
  Data Type Conversion : DataTypeConversion  OutDataTypeStr=uint8
  Data Type Conversion3 : DataTypeConversion
  Data Type Conversion8 : DataTypeConversion
  Demux1 : Demux  Outputs=1
  SPI_Master_Transfer_To1 : mbd_mpc574x_ec_toolbox/Communication Blocks/SPI Blocks/SPI_Master_Transfer  Priority=2  InstanceNumber=0  xfermode=Non blocking  timeout=50  spi_upd=on  WhichPCS=0
  Terminator : Terminator
  Vector Concatenate1 : Concatenate  NumInputs=1
  write_enable : Constant  Value=6  OutDataTypeStr=uint8
  wires:
  Data Type Conversion3/1 -> Terminator/1  "r8"
  SPI_Master_Transfer_To1/1 -> Demux1/1
  Demux1/1 -> Data Type Conversion3/1
  Vector Concatenate1/1 -> SPI_Master_Transfer_To1/1
  write_enable/1 -> Data Type Conversion/1
  Data Type Conversion/1 -> Vector Concatenate1/1  "d8"
  Constant1/1 -> Data Type Conversion8/1
  Data Type Conversion8/1 -> Data Store Write/1

== system ZT_VehCtrl_18B_CAN/SPI_EEPROM/SPI_write/SPI_write ==
  Action Port : ActionPort
  "Address_High " : Constant  Value=hex2dec('FF')  OutDataTypeStr=uint8
  Address_Low : Constant  Value=hex2dec('FF')
  Constant1 : Constant
  Data Store Read : DataStoreRead  DataStoreName=A_write
  Data Store Write : DataStoreWrite  DataStoreName=Write_Ctrl
  Data Type Conversion{,1..2,5} (4 alike) : DataTypeConversion  OutDataTypeStr=uint8
  Data Type Conversion{3..4,6..8} (5 alike) : DataTypeConversion
  Demux1 : Demux
  SPI_Master_Transfer_To1 : mbd_mpc574x_ec_toolbox/Communication Blocks/SPI Blocks/SPI_Master_Transfer  Priority=2  InstanceNumber=0  xfermode=Non blocking  timeout=50  spi_upd=on  WhichPCS=0
  Terminator{,1..3} (4 alike) : Terminator
  Vector Concatenate1 : Concatenate  NumInputs=4
  write_set : Constant  Value=2  OutDataTypeStr=uint8
  wires:
  Data Type Conversion4/1 -> Terminator1/1  "r5"
  Data Type Conversion3/1 -> Terminator/1  "r4"
  SPI_Master_Transfer_To1/1 -> Demux1/1
  Demux1/1 -> Data Type Conversion3/1
  Vector Concatenate1/1 -> SPI_Master_Transfer_To1/1
  Demux1/2 -> Data Type Conversion4/1
  Address_Low/1 -> Data Type Conversion5/1
  Data Type Conversion/1 -> Vector Concatenate1/1  "d4"
  Data Type Conversion1/1 -> Vector Concatenate1/2  "d5"
  write_set/1 -> Data Type Conversion/1
  "Address_High "/1 -> Data Type Conversion1/1
  Data Store Read/1 -> Data Type Conversion2/1
  Constant1/1 -> Data Type Conversion8/1
  Data Type Conversion5/1 -> Vector Concatenate1/3  "d6"
  Data Type Conversion2/1 -> Vector Concatenate1/4  "d7"
  Data Type Conversion6/1 -> Terminator2/1  "r6"
  Demux1/3 -> Data Type Conversion6/1
  Data Type Conversion7/1 -> Terminator3/1  "r7"
  Demux1/4 -> Data Type Conversion7/1
  Data Type Conversion8/1 -> Data Store Write/1

== system ZT_VehCtrl_18B_CAN/SigIn/CAN0 / BMS Power Control ==
  ID : Inport
  Data : Inport  Port=2
  length : Inport  Port=3
  timestamp : Inport  Port=4
  Switch Case : SwitchCase  CaseConditions={hex2dec('1F3')}  ShowDefaultCase=off
  UNPACK : Subsystem  TreatAsAtomicUnit=on
  Message : Outport
  wires:
  Switch Case/1 -> UNPACK/Action
  ID/1 -> UNPACK/1(ID), Switch Case/1
  Data/1 -> UNPACK/2(data)
  timestamp/1 -> UNPACK/4(timestamp)
  length/1 -> UNPACK/3(length)
  UNPACK/1(Message) -> Message/1

== system ZT_VehCtrl_18B_CAN/SigIn/CAN0 /ACU1 ==
  ID : Inport
  Data : Inport  Port=2
  length : Inport  Port=3
  timestamp : Inport  Port=4
  Switch Case : SwitchCase  CaseConditions={hex2dec('0C08A79A')}  ShowDefaultCase=off
  UNPACK : Subsystem  TreatAsAtomicUnit=on
  Message : Outport
  wires:
  Switch Case/1 -> UNPACK/Action
  ID/1 -> UNPACK/1(ID), Switch Case/1
  Data/1 -> UNPACK/2(data)
  timestamp/1 -> UNPACK/4(timestamp)
  length/1 -> UNPACK/3(length)
  UNPACK/1(Message) -> Message/1

== system ZT_VehCtrl_18B_CAN/SigIn/CAN0 /ACU2 ==
  ID : Inport
  Data : Inport  Port=2
  length : Inport  Port=3
  timestamp : Inport  Port=4
  Switch Case : SwitchCase  CaseConditions={hex2dec('0C09A79B')}  ShowDefaultCase=off
  UNPACK : Subsystem  TreatAsAtomicUnit=on
  Message : Outport
  wires:
  UNPACK/1(Message) -> Message/1
  length/1 -> UNPACK/3(length)
  timestamp/1 -> UNPACK/4(timestamp)
  Data/1 -> UNPACK/2(data)
  ID/1 -> Switch Case/1, UNPACK/1(ID)
  Switch Case/1 -> UNPACK/Action

== system ZT_VehCtrl_18B_CAN/SigIn/CAN0 /ACU3 ==
  ID : Inport
  Data : Inport  Port=2
  length : Inport  Port=3
  timestamp : Inport  Port=4
  Switch Case : SwitchCase  CaseConditions={hex2dec('0C0AA79D')}  ShowDefaultCase=off
  UNPACK : Subsystem  TreatAsAtomicUnit=on
  Message : Outport
  wires:
  Switch Case/1 -> UNPACK/Action
  ID/1 -> UNPACK/1(ID), Switch Case/1
  Data/1 -> UNPACK/2(data)
  timestamp/1 -> UNPACK/4(timestamp)
  length/1 -> UNPACK/3(length)
  UNPACK/1(Message) -> Message/1

== system ZT_VehCtrl_18B_CAN/SigIn/CAN0 /BMS Cell Battery Temperature ==
  ID : Inport
  Data : Inport  Port=2
  length : Inport  Port=3
  timestamp : Inport  Port=4
  Switch Case : SwitchCase  CaseConditions={hex2dec('357')}  ShowDefaultCase=off
  UNPACK : Subsystem  TreatAsAtomicUnit=on
  Message : Outport
  wires:
  UNPACK/1(Message) -> Message/1
  length/1 -> UNPACK/3(length)
  timestamp/1 -> UNPACK/4(timestamp)
  Data/1 -> UNPACK/2(data)
  ID/1 -> Switch Case/1, UNPACK/1(ID)
  Switch Case/1 -> UNPACK/Action

== system ZT_VehCtrl_18B_CAN/SigIn/CAN0 /BMS Cell HeatingTemperature ==
  ID : Inport
  Data : Inport  Port=2
  length : Inport  Port=3
  timestamp : Inport  Port=4
  Switch Case : SwitchCase  CaseConditions={hex2dec('3F3')}  ShowDefaultCase=off
  UNPACK : Subsystem  TreatAsAtomicUnit=on
  Message : Outport
  wires:
  Switch Case/1 -> UNPACK/Action
  ID/1 -> UNPACK/1(ID), Switch Case/1
  Data/1 -> UNPACK/2(data)
  timestamp/1 -> UNPACK/4(timestamp)
  length/1 -> UNPACK/3(length)
  UNPACK/1(Message) -> Message/1

== system ZT_VehCtrl_18B_CAN/SigIn/CAN0 /BMS Cell Pole Temperature ==
  ID : Inport
  Data : Inport  Port=2
  length : Inport  Port=3
  timestamp : Inport  Port=4
  Switch Case : SwitchCase  CaseConditions={hex2dec('3F4')}  ShowDefaultCase=off
  UNPACK : Subsystem  TreatAsAtomicUnit=on
  Message : Outport
  wires:
  UNPACK/1(Message) -> Message/1
  length/1 -> UNPACK/3(length)
  timestamp/1 -> UNPACK/4(timestamp)
  Data/1 -> UNPACK/2(data)
  ID/1 -> Switch Case/1, UNPACK/1(ID)
  Switch Case/1 -> UNPACK/Action

== system ZT_VehCtrl_18B_CAN/SigIn/CAN0 /BMS Cell Voltage Infor ==
  ID : Inport
  Data : Inport  Port=2
  length : Inport  Port=3
  timestamp : Inport  Port=4
  Switch Case : SwitchCase  CaseConditions={hex2dec('356')}  ShowDefaultCase=off
  UNPACK : Subsystem  TreatAsAtomicUnit=on
  Message : Outport
  wires:
  UNPACK/1(Message) -> Message/1
  length/1 -> UNPACK/3(length)
  timestamp/1 -> UNPACK/4(timestamp)
  Data/1 -> UNPACK/2(data)
  ID/1 -> Switch Case/1, UNPACK/1(ID)
  Switch Case/1 -> UNPACK/Action

== system ZT_VehCtrl_18B_CAN/SigIn/CAN0 /BMS CumuCap Infor ==
  ID : Inport
  Data : Inport  Port=2
  length : Inport  Port=3
  timestamp : Inport  Port=4
  Switch Case : SwitchCase  CaseConditions={hex2dec('3F5')}  ShowDefaultCase=off
  UNPACK : Subsystem  TreatAsAtomicUnit=on
  Message : Outport
  wires:
  Switch Case/1 -> UNPACK/Action
  ID/1 -> UNPACK/1(ID), Switch Case/1
  Data/1 -> UNPACK/2(data)
  timestamp/1 -> UNPACK/4(timestamp)
  length/1 -> UNPACK/3(length)
  UNPACK/1(Message) -> Message/1

== system ZT_VehCtrl_18B_CAN/SigIn/CAN0 /BMS CumuTimeInfor1 ==
  ID : Inport
  Data : Inport  Port=2
  length : Inport  Port=3
  timestamp : Inport  Port=4
  Switch Case : SwitchCase  CaseConditions={hex2dec('203')}  ShowDefaultCase=off
  UNPACK : Subsystem  TreatAsAtomicUnit=on
  Message : Outport
  wires:
  UNPACK/1(Message) -> Message/1
  length/1 -> UNPACK/3(length)
  timestamp/1 -> UNPACK/4(timestamp)
  Data/1 -> UNPACK/2(data)
  ID/1 -> Switch Case/1, UNPACK/1(ID)
  Switch Case/1 -> UNPACK/Action

== system ZT_VehCtrl_18B_CAN/SigIn/CAN0 /BMS CumuTimeInfor2 ==
  ID : Inport
  Data : Inport  Port=2
  length : Inport  Port=3
  timestamp : Inport  Port=4
  Switch Case : SwitchCase  CaseConditions={hex2dec('204')}  ShowDefaultCase=off
  UNPACK : Subsystem  TreatAsAtomicUnit=on
  Message : Outport
  wires:
  Switch Case/1 -> UNPACK/Action
  ID/1 -> UNPACK/1(ID), Switch Case/1
  Data/1 -> UNPACK/2(data)
  timestamp/1 -> UNPACK/4(timestamp)
  length/1 -> UNPACK/3(length)
  UNPACK/1(Message) -> Message/1

== system ZT_VehCtrl_18B_CAN/SigIn/CAN0 /BMS HeatInfor ==
  ID : Inport
  Data : Inport  Port=2
  length : Inport  Port=3
  timestamp : Inport  Port=4
  Switch Case : SwitchCase  CaseConditions={hex2dec('208')}  ShowDefaultCase=off
  UNPACK : Subsystem  TreatAsAtomicUnit=on
  Message : Outport
  wires:
  Switch Case/1 -> UNPACK/Action
  ID/1 -> UNPACK/1(ID), Switch Case/1
  Data/1 -> UNPACK/2(data)
  timestamp/1 -> UNPACK/4(timestamp)
  length/1 -> UNPACK/3(length)
  UNPACK/1(Message) -> Message/1

== system ZT_VehCtrl_18B_CAN/SigIn/CAN0 /BMS Power Infor ==
  ID : Inport
  Data : Inport  Port=2
  length : Inport  Port=3
  timestamp : Inport  Port=4
  Switch Case : SwitchCase  CaseConditions={hex2dec('211')}  ShowDefaultCase=off
  UNPACK : Subsystem  TreatAsAtomicUnit=on
  Message : Outport
  wires:
  Switch Case/1 -> UNPACK/Action
  ID/1 -> UNPACK/1(ID), Switch Case/1
  Data/1 -> UNPACK/2(data)
  timestamp/1 -> UNPACK/4(timestamp)
  length/1 -> UNPACK/3(length)
  UNPACK/1(Message) -> Message/1

== system ZT_VehCtrl_18B_CAN/SigIn/CAN0 /BMS StartDia_Infor1 ==
  ID : Inport
  Data : Inport  Port=2
  length : Inport  Port=3
  timestamp : Inport  Port=4
  Switch Case : SwitchCase  CaseConditions={hex2dec('206')}  ShowDefaultCase=off
  UNPACK : Subsystem  TreatAsAtomicUnit=on
  Message : Outport
  wires:
  Switch Case/1 -> UNPACK/Action
  ID/1 -> UNPACK/1(ID), Switch Case/1
  Data/1 -> UNPACK/2(data)
  timestamp/1 -> UNPACK/4(timestamp)
  length/1 -> UNPACK/3(length)
  UNPACK/1(Message) -> Message/1

== system ZT_VehCtrl_18B_CAN/SigIn/CAN0 /BMS StartDia_Infor2 ==
  ID : Inport
  Data : Inport  Port=2
  length : Inport  Port=3
  timestamp : Inport  Port=4
  Switch Case : SwitchCase  CaseConditions={hex2dec('207')}  ShowDefaultCase=off
  UNPACK : Subsystem  TreatAsAtomicUnit=on
  Message : Outport
  wires:
  UNPACK/1(Message) -> Message/1
  length/1 -> UNPACK/3(length)
  timestamp/1 -> UNPACK/4(timestamp)
  Data/1 -> UNPACK/2(data)
  ID/1 -> Switch Case/1, UNPACK/1(ID)
  Switch Case/1 -> UNPACK/Action

== system ZT_VehCtrl_18B_CAN/SigIn/CAN0 /BMS Statistic_Cell ExtremumIndex Infor ==
  ID : Inport
  Data : Inport  Port=2
  length : Inport  Port=3
  timestamp : Inport  Port=4
  Switch Case : SwitchCase  CaseConditions={hex2dec('358')}  ShowDefaultCase=off
  UNPACK : Subsystem  TreatAsAtomicUnit=on
  Message : Outport
  wires:
  UNPACK/1(Message) -> Message/1
  length/1 -> UNPACK/3(length)
  timestamp/1 -> UNPACK/4(timestamp)
  Data/1 -> UNPACK/2(data)
  ID/1 -> Switch Case/1, UNPACK/1(ID)
  Switch Case/1 -> UNPACK/Action

== system ZT_VehCtrl_18B_CAN/SigIn/CAN0 /BMS Statistic_Cell Voltage Infor ==
  ID : Inport
  Data : Inport  Port=2
  length : Inport  Port=3
  timestamp : Inport  Port=4
  Switch Case : SwitchCase  CaseConditions={hex2dec('352')}  ShowDefaultCase=off
  UNPACK : Subsystem  TreatAsAtomicUnit=on
  Message : Outport
  wires:
  UNPACK/1(Message) -> Message/1
  length/1 -> UNPACK/3(length)
  timestamp/1 -> UNPACK/4(timestamp)
  Data/1 -> UNPACK/2(data)
  ID/1 -> Switch Case/1, UNPACK/1(ID)
  Switch Case/1 -> UNPACK/Action

== system ZT_VehCtrl_18B_CAN/SigIn/CAN0 /BMS Statistic_HeatingTemperature ==
  ID : Inport
  Data : Inport  Port=2
  length : Inport  Port=3
  timestamp : Inport  Port=4
  Switch Case : SwitchCase  CaseConditions={hex2dec('354')}  ShowDefaultCase=off
  UNPACK : Subsystem  TreatAsAtomicUnit=on
  Message : Outport
  wires:
  UNPACK/1(Message) -> Message/1
  length/1 -> UNPACK/3(length)
  timestamp/1 -> UNPACK/4(timestamp)
  Data/1 -> UNPACK/2(data)
  ID/1 -> Switch Case/1, UNPACK/1(ID)
  Switch Case/1 -> UNPACK/Action

== system ZT_VehCtrl_18B_CAN/SigIn/CAN0 /BMS Statistic_PoleTemperature ==
  ID : Inport
  Data : Inport  Port=2
  length : Inport  Port=3
  timestamp : Inport  Port=4
  Switch Case : SwitchCase  CaseConditions={hex2dec('355')}  ShowDefaultCase=off
  UNPACK : Subsystem  TreatAsAtomicUnit=on
  Message : Outport
  wires:
  UNPACK/1(Message) -> Message/1
  length/1 -> UNPACK/3(length)
  timestamp/1 -> UNPACK/4(timestamp)
  Data/1 -> UNPACK/2(data)
  ID/1 -> Switch Case/1, UNPACK/1(ID)
  Switch Case/1 -> UNPACK/Action

== system ZT_VehCtrl_18B_CAN/SigIn/CAN0 /BMS Statistic_Temperature of Battery ==
  ID : Inport
  Data : Inport  Port=2
  length : Inport  Port=3
  timestamp : Inport  Port=4
  Switch Case : SwitchCase  CaseConditions={hex2dec('353')}  ShowDefaultCase=off
  UNPACK : Subsystem  TreatAsAtomicUnit=on
  Message : Outport
  wires:
  UNPACK/1(Message) -> Message/1
  length/1 -> UNPACK/3(length)
  timestamp/1 -> UNPACK/4(timestamp)
  Data/1 -> UNPACK/2(data)
  ID/1 -> Switch Case/1, UNPACK/1(ID)
  Switch Case/1 -> UNPACK/Action

== system ZT_VehCtrl_18B_CAN/SigIn/CAN0 /BMS _SystemTime  ==
  ID : Inport
  Data : Inport  Port=2
  length : Inport  Port=3
  timestamp : Inport  Port=4
  Switch Case : SwitchCase  CaseConditions={hex2dec('202')}  ShowDefaultCase=off
  UNPACK : Subsystem  TreatAsAtomicUnit=on
  Message : Outport
  wires:
  Switch Case/1 -> UNPACK/Action
  ID/1 -> UNPACK/1(ID), Switch Case/1
  Data/1 -> UNPACK/2(data)
  timestamp/1 -> UNPACK/4(timestamp)
  length/1 -> UNPACK/3(length)
  UNPACK/1(Message) -> Message/1

== system ZT_VehCtrl_18B_CAN/SigIn/CAN0 /BMS other Information1 ==
  ID : Inport
  Data : Inport  Port=2
  length : Inport  Port=3
  timestamp : Inport  Port=4
  Switch Case : SwitchCase  CaseConditions={hex2dec('3F6')}  ShowDefaultCase=off
  UNPACK : Subsystem  TreatAsAtomicUnit=on
  Message : Outport
  wires:
  UNPACK/1(Message) -> Message/1
  length/1 -> UNPACK/3(length)
  timestamp/1 -> UNPACK/4(timestamp)
  Data/1 -> UNPACK/2(data)
  ID/1 -> Switch Case/1, UNPACK/1(ID)
  Switch Case/1 -> UNPACK/Action

== system ZT_VehCtrl_18B_CAN/SigIn/CAN0 /BMS other Information2  ==
  ID : Inport
  Data : Inport  Port=2
  length : Inport  Port=3
  timestamp : Inport  Port=4
  Switch Case : SwitchCase  CaseConditions={hex2dec('3FF')}  ShowDefaultCase=off
  UNPACK : Subsystem  TreatAsAtomicUnit=on
  Message : Outport
  wires:
  Switch Case/1 -> UNPACK/Action
  ID/1 -> UNPACK/1(ID), Switch Case/1
  Data/1 -> UNPACK/2(data)
  timestamp/1 -> UNPACK/4(timestamp)
  length/1 -> UNPACK/3(length)
  UNPACK/1(Message) -> Message/1

== system ZT_VehCtrl_18B_CAN/SigIn/CAN0 /BMS other Information3 ==
  ID : Inport
  Data : Inport  Port=2
  length : Inport  Port=3
  timestamp : Inport  Port=4
  Switch Case : SwitchCase  CaseConditions={hex2dec('205')}  ShowDefaultCase=off
  UNPACK : Subsystem  TreatAsAtomicUnit=on
  Message : Outport
  wires:
  UNPACK/1(Message) -> Message/1
  length/1 -> UNPACK/3(length)
  timestamp/1 -> UNPACK/4(timestamp)
  Data/1 -> UNPACK/2(data)
  ID/1 -> Switch Case/1, UNPACK/1(ID)
  Switch Case/1 -> UNPACK/Action

== system ZT_VehCtrl_18B_CAN/SigIn/CAN0 /BMSWarning_Status ==
  ID : Inport
  Data : Inport  Port=2
  length : Inport  Port=3
  timestamp : Inport  Port=4
  Switch Case : SwitchCase  CaseConditions={hex2dec('1F5')}  ShowDefaultCase=off
  UNPACK : Subsystem  TreatAsAtomicUnit=on
  Message : Outport
  wires:
  UNPACK/1(Message) -> Message/1
  length/1 -> UNPACK/3(length)
  timestamp/1 -> UNPACK/4(timestamp)
  Data/1 -> UNPACK/2(data)
  ID/1 -> Switch Case/1, UNPACK/1(ID)
  Switch Case/1 -> UNPACK/Action

== system ZT_VehCtrl_18B_CAN/SigIn/CAN0 /BMS_Information1 ==
  ID : Inport
  Data : Inport  Port=2
  length : Inport  Port=3
  timestamp : Inport  Port=4
  Switch Case : SwitchCase  CaseConditions={hex2dec('1E1')}  ShowDefaultCase=off
  UNPACK : Subsystem  TreatAsAtomicUnit=on
  Message : Outport
  wires:
  UNPACK/1(Message) -> Message/1
  length/1 -> UNPACK/3(length)
  timestamp/1 -> UNPACK/4(timestamp)
  Data/1 -> UNPACK/2(data)
  ID/1 -> Switch Case/1, UNPACK/1(ID)
  Switch Case/1 -> UNPACK/Action

== system ZT_VehCtrl_18B_CAN/SigIn/CAN0 /BMS_Information2 ==
  ID : Inport
  Data : Inport  Port=2
  length : Inport  Port=3
  timestamp : Inport  Port=4
  Switch Case : SwitchCase  CaseConditions={hex2dec('1E4')}  ShowDefaultCase=off
  UNPACK : Subsystem  TreatAsAtomicUnit=on
  Message : Outport
  wires:
  Switch Case/1 -> UNPACK/Action
  ID/1 -> UNPACK/1(ID), Switch Case/1
  Data/1 -> UNPACK/2(data)
  timestamp/1 -> UNPACK/4(timestamp)
  length/1 -> UNPACK/3(length)
  UNPACK/1(Message) -> Message/1

== system ZT_VehCtrl_18B_CAN/SigIn/CAN0 /BMS_Relay Status1 ==
  ID : Inport
  Data : Inport  Port=2
  length : Inport  Port=3
  timestamp : Inport  Port=4
  Switch Case : SwitchCase  CaseConditions={hex2dec('351')}  ShowDefaultCase=off
  UNPACK : Subsystem  TreatAsAtomicUnit=on
  Message : Outport
  wires:
  UNPACK/1(Message) -> Message/1
  length/1 -> UNPACK/3(length)
  timestamp/1 -> UNPACK/4(timestamp)
  Data/1 -> UNPACK/2(data)
  ID/1 -> Switch Case/1, UNPACK/1(ID)
  Switch Case/1 -> UNPACK/Action

== system ZT_VehCtrl_18B_CAN/SigIn/CAN0 /BMS_Relay Status2 ==
  ID : Inport
  Data : Inport  Port=2
  length : Inport  Port=3
  timestamp : Inport  Port=4
  Switch Case : SwitchCase  CaseConditions={hex2dec('360')}  ShowDefaultCase=off
  UNPACK : Subsystem  TreatAsAtomicUnit=on
  Message : Outport
  wires:
  UNPACK/1(Message) -> Message/1
  length/1 -> UNPACK/3(length)
  timestamp/1 -> UNPACK/4(timestamp)
  Data/1 -> UNPACK/2(data)
  ID/1 -> Switch Case/1, UNPACK/1(ID)
  Switch Case/1 -> UNPACK/Action

== system ZT_VehCtrl_18B_CAN/SigIn/CAN0 /BMS_Relay Status3 ==
  ID : Inport
  Data : Inport  Port=2
  length : Inport  Port=3
  timestamp : Inport  Port=4
  Switch Case : SwitchCase  CaseConditions={hex2dec('361')}  ShowDefaultCase=off
  UNPACK : Subsystem  TreatAsAtomicUnit=on
  Message : Outport
  wires:
  Switch Case/1 -> UNPACK/Action
  ID/1 -> UNPACK/1(ID), Switch Case/1
  Data/1 -> UNPACK/2(data)
  timestamp/1 -> UNPACK/4(timestamp)
  length/1 -> UNPACK/3(length)
  UNPACK/1(Message) -> Message/1
